simulink model "carsim_with_simulink3dof_open_loop_specific_control"  (R2023b)
settings: Solver=FixedStepAuto  StartTime=0.0  StopTime=25  FixedStep=0.001  RelTol=1e-3  EnableMultiTasking=on
values from neighbouring files (symbols this model uses):
  A = 5    [unlinear_vehicle_Parameters.m]
  Bf = 1.725    [unlinear_vehicle_Parameters.m]
  Br = 1.750    (= 1.75)    [unlinear_vehicle_Parameters.m]
  Cd = 0.4    [unlinear_vehicle_Parameters.m]
  Cs_f = 4302    [unlinear_vehicle_Parameters.m]
  Delta_act_sine_amp = delta_act_sine_amp(j)    [Truck_simulate.m]    (also in unlinear_vehicle_Parameters.m)
  Delta_act_sine_fre = delta_act_sine_fre(k)    [Truck_simulate.m]    (also in unlinear_vehicle_Parameters.m)
  f = 0.01    [unlinear_vehicle_Parameters.m]
  g = 9.8    [Truck_simulate.m]    (also in unlinear_vehicle_Parameters.m)
  He = 0.45    [unlinear_vehicle_Parameters.m]
  hg = 0.781    [unlinear_vehicle_Parameters.m]
  Hp = 0.2    [unlinear_vehicle_Parameters.m]
  I_tire = 0.7    [unlinear_vehicle_Parameters.m]
  Ix = 423.3    [unlinear_vehicle_Parameters.m]
  Iy = 1762.5    [unlinear_vehicle_Parameters.m]
  Iz = 1762.5    [unlinear_vehicle_Parameters.m]
  ks_f = 189000    [unlinear_vehicle_Parameters.m]
  kw = 220000    [unlinear_vehicle_Parameters.m]
  L = 3.140    (= 3.14)    [unlinear_vehicle_Parameters.m]
  Lf = 1.330    (= 1.33)    [unlinear_vehicle_Parameters.m]
  Lr = 3.140 - 1.330    (= 1.81)    [unlinear_vehicle_Parameters.m]
  m = m_sprung + m_load + m_unsprung    (= 10505)    [Truck_simulate.m]    (also in unlinear_vehicle_Parameters.m = 1407.3)
  mb = 1128.5 + 000    (= 1128.5)    [unlinear_vehicle_Parameters.m]
  mw = 139.4 / 2    (= 69.7)    [unlinear_vehicle_Parameters.m]
  p = 1.206    [unlinear_vehicle_Parameters.m]
  r = 0.510    (= 0.51)    [Truck_simulate.m]    (also in unlinear_vehicle_Parameters.m = 0.287)
  T_motor_constant = t_motor_const(i)    [Truck_simulate.m]    (also in unlinear_vehicle_Parameters.m)
  vx0 = 5    [Truck_simulate.m]    (also in unlinear_vehicle_Parameters.m)
  vy0 = 0    [Truck_simulate.m]    (also in unlinear_vehicle_Parameters.m)
  w0 = vx0 / r    (= 9.80392156863)    [Truck_simulate.m]    (also in unlinear_vehicle_Parameters.m = 17.4216027875)
  wz0 = 0    [Truck_simulate.m]    (also in unlinear_vehicle_Parameters.m)
libraries: Solver_SF x1
(part 1 of 4)
settings Model: Creator=dzY  LastModifiedBy=Admin
settings SolverCC: AlgebraicLoopSolver=TrustRegion
settings DataIOCC: SaveFormat=Array  ReturnWorkspaceOutputs=off
settings OptimizationCC: LifeSpan=inf
settings DebuggingCC: SolverPrmCheckMsg=warning  UnconnectedInputMsg=warning  UnconnectedOutputMsg=warning  UnconnectedLineMsg=warning  SFUnexpectedBacktrackingDiag=warning  SFNoUnconditionalDefaultTransitionDiag=warning  SFExecutionAtInitializationDiag=none  ArithmeticOperatorsInVariantConditions=warning
settings HardwareCC: ProdBitPerPointer=32  ProdBitPerSizeT=32  ProdBitPerPtrDiffT=32  ProdLargestAtomicFloat=None  ProdIntDivRoundTo=Undefined  ProdEndianess=Unspecified  ProdWordSize=32  ProdHWDeviceType=32-bit Generic
settings ModelReferenceCC: EnableRefExpFcnMdlSchedulingChecks=on  PropagateSignalLabelsOutOfModel=off
settings SFSimCC: SimUseLocalCustomCode=off  CustomCodeUndefinedFunction=UseInterfaceOnly
settings RTWCC: RTWUseLocalCustomCode=off
settings CodeAppCC: StateflowObjectComments=on
settings GRTTargetCC: TargetLangStandard=C89/C90 (ANSI)
settings ConfigComp: CovMetricSettings=dw  CovSaveCumulativeToWorkspaceVar=on  CovSaveSingleToWorkspaceVar=on  CovExternalEMLEnable=off  CovSFcnEnable=off

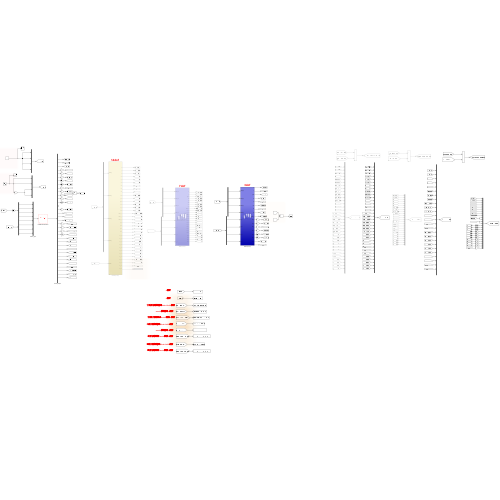
[thumbnail: Simulink's stored preview of the top-level diagram]
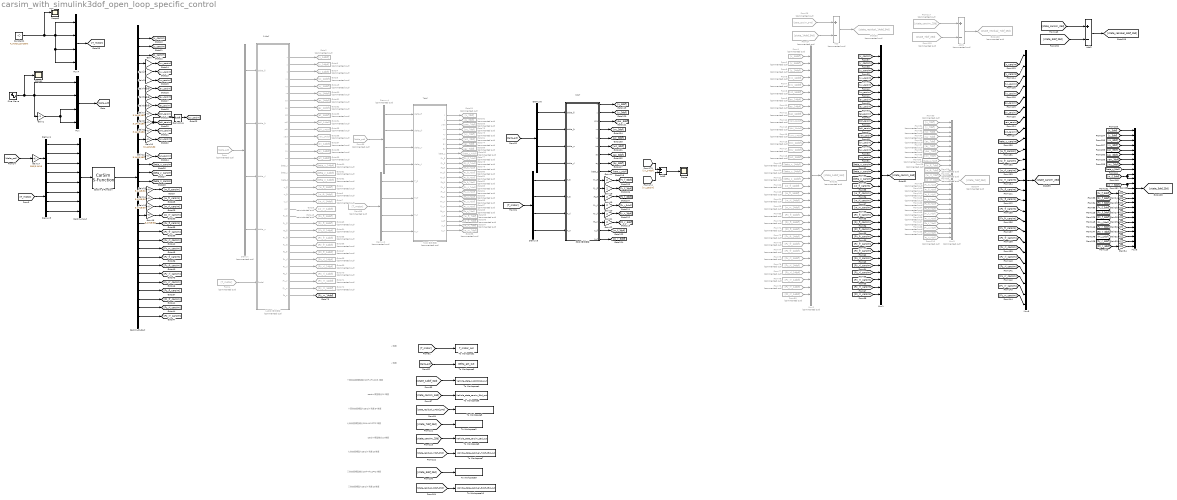
== system carsim_with_simulink3dof_open_loop_specific_control ==
  note: 7dof
  note: 4维度
  note: 4维度
  note: 十四自由度模型输出18+4+12=34维度
  note: carsim模型输出34维度
  note: 十四自由度模型与carsim残差34维度
  note: carsim模型输出25维度
  note: 七自由度模型与carsim残差25维度
  note: 七自由度模型输出18+4+12=25维度
  note: 14dof
  note: 3dof
  note: 三自由度模型与carsim残差25维度
  note: 三自由度模型输出18+4+12=25维度
  14DOF整车模型 : Subsystem  Commented=on
  3DOF整车模型 : Subsystem
  7DOF整车模型 : Subsystem  Commented=on
  Add : Sum  Commented=on  Inputs=+-
  Add1 : Sum  Commented=on  Inputs=+-
  Add2 : Sum  Inputs=+-
  Add3 : Sum  Inputs=+-
  CarSim S-Function : Solver_SF/CarSim S-Function  Priority=1  SIMFILE=simfile.sim  Run_RTs=off  vs_state_ind=Run  StopMode_ind=Vehicle Model
  Carsim_Input : Mux  Inputs=8
  Carsim_Output : Demux  Outputs=34
  Constant1 : Constant  Value=T_motor_constant
  Demux : Demux  Commented=on
  Demux{1,3,5..6} (4 alike) : Demux
  Demux2 : Demux  Commented=on
  Demux4 : Demux  Commented=on
  Derivative : Derivative
  From : From  Commented=on  GotoTag=delta_act
  From1 : From  Commented=on  GotoTag=x_14dof
  From10 : From  Commented=on  GotoTag=ay_14dof
  From100 : From  Commented=on  GotoTag=Fy_fl_7dof
  From101 : From  Commented=on  GotoTag=Fz_fl_7dof
  From102 : From  Commented=on  GotoTag=Fx_fr_7dof
  From103 : From  Commented=on  GotoTag=Fy_fr_7dof
  From104 : From  Commented=on  GotoTag=Fz_fr_7dof
  From105 : From  Commented=on  GotoTag=Fx_rl_7dof
  From106 : From  Commented=on  GotoTag=Fy_rl_7dof
  From107 : From  Commented=on  GotoTag=Fz_rl_7dof
  From108 : From  Commented=on  GotoTag=Fx_rr_7dof
  From109 : From  Commented=on  GotoTag=Fy_rr_7dof
  From11 : From  Commented=on  GotoTag=az_14dof
  From110 : From  Commented=on  GotoTag=Fz_rr_7dof
  From115 : From  Commented=on  GotoTag=state_7dof_25d
  From117 : From  Commented=on  GotoTag=state_carsim_25d
  From12 : From  Commented=on  GotoTag=roll_14dof
  From13 : From  Commented=on  GotoTag=phi_14dof
  From15 : From  Commented=on  GotoTag=yaw_14dof
  From16 : From  Commented=on  GotoTag=wx_14dof
  From17 : From  Commented=on  GotoTag=wy_14dof
  From18 : From  Commented=on  GotoTag=wz_14dof
  From19 : From  Commented=on  GotoTag=beta_x_14dof
  From2 : From  Commented=on  GotoTag=y_14dof
  From20 : From  Commented=on  GotoTag=beta_y_14dof
  From21 : From  Commented=on  GotoTag=beta_z_14dof
  From22 : From  Commented=on  GotoTag=w_fl_14dof
  From23 : From  Commented=on  GotoTag=w_fr_14dof
  From24 : From  Commented=on  GotoTag=w_rl_14dof
  From25 : From  Commented=on  GotoTag=w_rr_14dof
  From26 : From  Commented=on  GotoTag=state_carsim_34d
  From27 : From  Commented=on  GotoTag=state_14dof_34d
  From28 : From  Commented=on  GotoTag=w_fl_7dof
  From29 : From  Commented=on  GotoTag=w_fr_7dof
  From30 : From  Commented=on  GotoTag=w_rl_7dof
  From4 : From  Commented=on  GotoTag=T_motor
  From5 : From  Commented=on  GotoTag=z_14dof
  From6 : From  Commented=on  GotoTag=vx_14dof
  From69 : From  Commented=on  GotoTag=Fx_fl_14dof
  From7 : From  Commented=on  GotoTag=vy_14dof
  From70 : From  Commented=on  GotoTag=Fy_fl_14dof
  From71 : From  Commented=on  GotoTag=Fz_fl_14dof
  From72 : From  Commented=on  GotoTag=Fx_fr_14dof
  From73 : From  Commented=on  GotoTag=Fy_fr_14dof
  From74 : From  Commented=on  GotoTag=Fz_fr_14dof
  From75 : From  Commented=on  GotoTag=Fx_rl_14dof
  From76 : From  Commented=on  GotoTag=Fy_rl_14dof
  From77 : From  Commented=on  GotoTag=Fz_rl_14dof
  From78 : From  Commented=on  GotoTag=Fx_rr_14dof
  From79 : From  Commented=on  GotoTag=Fy_rr_14dof
  From8 : From  Commented=on  GotoTag=vz_14dof
  From80 : From  Commented=on  GotoTag=Fz_rr_14dof
  From85 : From  Commented=on  GotoTag=w_rr_7dof
  From88 : From  Commented=on  GotoTag=T_motor
  From89 : From  Commented=on  GotoTag=delta_act
  From9 : From  Commented=on  GotoTag=ax_14dof
  From90 : From  Commented=on  GotoTag=x_7dof
  From91 : From  Commented=on  GotoTag=y_7dof
  From92 : From  Commented=on  GotoTag=yaw_7dof
  From93 : From  Commented=on  GotoTag=vx_7dof
  From94 : From  Commented=on  GotoTag=vy_7dof
  From95 : From  Commented=on  GotoTag=wz_7dof
  From96 : From  Commented=on  GotoTag=ax_7dof
  From97 : From  Commented=on  GotoTag=ay_7dof
  From98 : From  Commented=on  GotoTag=beta_z_7dof
  From99 : From  Commented=on  GotoTag=Fx_fl_7dof
  Gain : Gain  Gain=1/3.6
  Gain1 : Gain  Gain=-1
  Gain{7..10,12} (5 alike) : Gain  Gain=3.1415/180
  Gain{11,18..22} (6 alike) : Gain  Gain=2
  Gain{13..16} (4 alike) : Gain  Gain=3.1415/30
  Gain17 : Gain  Gain=180/3.1415
  Gain2 : Gain  Gain=1/3.6
  Gain{23..34} (12 alike) : Gain  Gain=0.5
  Gain3 : Gain  Gain=1/3.6
  Gain4 : Gain  Gain=9.8
  Gain5 : Gain  Gain=9.8
  Gain6 : Gain  Gain=9.8
  Goto1 : Goto  Commented=on  GotoTag=w_fl_14dof
  Goto100 : Goto  Commented=on  GotoTag=state_residual_7dof_25d
  Goto2 : Goto  Commented=on  GotoTag=x_14dof
  Goto3 : Goto  Commented=on  GotoTag=y_14dof
  Goto32 : Goto  Commented=on  GotoTag=state_14dof_34d
  Goto33 : Goto  Commented=on  GotoTag=state_residual_14dof_34d
  Goto34 : Goto  Commented=on  GotoTag=wz_7dof
  Goto4 : Goto  Commented=on  GotoTag=z_14dof
  Goto48 : Goto  Commented=on  GotoTag=Fx_fl_14dof
  Goto49 : Goto  Commented=on  GotoTag=vy_14dof
  Goto5 : Goto  Commented=on  GotoTag=vx_14dof
  Goto50 : Goto  Commented=on  GotoTag=vz_14dof
  Goto51 : Goto  Commented=on  GotoTag=ax_14dof
  Goto52 : Goto  Commented=on  GotoTag=ay_14dof
  Goto53 : Goto  Commented=on  GotoTag=az_14dof
  Goto54 : Goto  Commented=on  GotoTag=roll_14dof
  Goto55 : Goto  Commented=on  GotoTag=phi_14dof
  Goto56 : Goto  Commented=on  GotoTag=yaw_14dof
  Goto57 : Goto  Commented=on  GotoTag=wx_14dof
  Goto58 : Goto  Commented=on  GotoTag=wy_14dof
  Goto59 : Goto  Commented=on  GotoTag=wz_14dof
  Goto6 : Goto  Commented=on  GotoTag=w_fr_14dof
  Goto60 : Goto  Commented=on  GotoTag=beta_x_14dof
  Goto61 : Goto  Commented=on  GotoTag=beta_y_14dof
  Goto62 : Goto  Commented=on  GotoTag=beta_z_14dof
  Goto63 : Goto  Commented=on  GotoTag=Fy_fl_14dof
  Goto64 : Goto  Commented=on  GotoTag=Fz_fl_14dof
  Goto65 : Goto  Commented=on  GotoTag=Fx_fr_14dof
  Goto66 : Goto  Commented=on  GotoTag=Fy_fr_14dof
  Goto67 : Goto  Commented=on  GotoTag=Fz_fr_14dof
  Goto68 : Goto  Commented=on  GotoTag=Fx_rl_14dof
  Goto69 : Goto  Commented=on  GotoTag=Fy_rl_14dof
  Goto7 : Goto  Commented=on  GotoTag=w_rl_14dof
  Goto70 : Goto  Commented=on  GotoTag=Fz_rl_14dof
  Goto71 : Goto  Commented=on  GotoTag=Fx_rr_14dof
  Goto72 : Goto  Commented=on  GotoTag=Fy_rr_14dof
  Goto74 : Goto  Commented=on  GotoTag=ax_7dof
  Goto75 : Goto  Commented=on  GotoTag=vy_7dof
  Goto76 : Goto  Commented=on  GotoTag=vx_7dof
  Goto77 : Goto  Commented=on  GotoTag=Fx_fl_7dof
  Goto78 : Goto  Commented=on  GotoTag=Fy_fl_7dof
  Goto79 : Goto  Commented=on  GotoTag=Fz_fl_7dof
  Goto8 : Goto  Commented=on  GotoTag=w_rr_14dof
  Goto80 : Goto  Commented=on  GotoTag=Fx_fr_7dof
  Goto81 : Goto  Commented=on  GotoTag=Fy_fr_7dof
  Goto82 : Goto  Commented=on  GotoTag=Fz_fr_7dof
  Goto83 : Goto  Commented=on  GotoTag=Fx_rl_7dof
  Goto84 : Goto  Commented=on  GotoTag=Fy_rl_7dof
  Goto85 : Goto  Commented=on  GotoTag=Fz_rl_7dof
  Goto86 : Goto  Commented=on  GotoTag=Fx_rr_7dof
  Goto87 : Goto  Commented=on  GotoTag=Fy_rr_7dof
  Goto88 : Goto  Commented=on  GotoTag=Fz_rr_7dof
  Goto89 : Goto  Commented=on  GotoTag=ay_7dof
  Goto90 : Goto  Commented=on  GotoTag=beta_z_7dof
  Goto91 : Goto  Commented=on  GotoTag=x_7dof
  Goto92 : Goto  Commented=on  GotoTag=y_7dof
  Goto93 : Goto  Commented=on  GotoTag=yaw_7dof
  Goto94 : Goto  Commented=on  GotoTag=state_7dof_25d
  Goto95 : Goto  Commented=on  GotoTag=w_fl_7dof
  Goto96 : Goto  Commented=on  GotoTag=w_fr_7dof
  Goto97 : Goto  Commented=on  GotoTag=w_rl_7dof
  Goto98 : Goto  Commented=on  GotoTag=w_rr_7dof
  Mux : Mux
  Mux1 : Mux  Inputs=34
  Mux2 : Mux  Commented=on  Inputs=34
  Mux3 : Mux  Commented=on  Inputs=25
  Mux4 : Mux
  Mux5 : Mux  Inputs=25
  Mux6 : Mux  Inputs=25
  Scope : Scope
  Scope4 : Scope
  Scope5 : Scope
  Sine Wave : Sin  Amplitude=Delta_act_sine_amp  Frequency=Delta_act_sine_fre  SampleTime=0
  To Workspace1 : ToWorkspace  VariableName=T_motor_out  SaveFormat=Timeseries  SampleTime=-1
  To Workspace10 : ToWorkspace  VariableName=Vehicle_state_residual_3dof_25d_out  SaveFormat=Timeseries  SampleTime=-1
  To Workspace2 : ToWorkspace  VariableName=Vehicle_state_7dof_25d_out  SaveFormat=Timeseries  SampleTime=-1
  To Workspace3 : ToWorkspace  VariableName=Delta_act_out  SaveFormat=Timeseries  SampleTime=-1
  To Workspace4 : ToWorkspace  VariableName=Vehicle_state_14dof_34d_out  SaveFormat=Timeseries  SampleTime=-1
  To Workspace5 : ToWorkspace  VariableName=Vehicle_state_residual_14dof_34d_out  SaveFormat=Timeseries  SampleTime=-1
  To Workspace6 : ToWorkspace  VariableName=Vehicle_state_carsim_34d_out  SaveFormat=Timeseries  SampleTime=-1
  To Workspace7 : ToWorkspace  VariableName=Vehicle_state_residual_7dof_25d_out  SaveFormat=Timeseries  SampleTime=-1
  To Workspace8 : ToWorkspace  VariableName=Vehicle_state_carsim_25d_out  SaveFormat=Timeseries  SampleTime=-1
  To Workspace9 : ToWorkspace  VariableName=Vehicle_state_3dof_25d_out  SaveFormat=Timeseries  SampleTime=-1
  wires:
  From4/1 -> 14DOF整车模型/5(Pedal)
  Mux4/1 -> [T_motor]
  Constant1/1 -> Mux4/1, Mux4/4, Mux4/3, Mux4/2, Scope5/1
  Carsim_Input/1 -> CarSim S-Function/1
  CarSim S-Function/1 -> Carsim_Output/1
  [T_motor] -> Demux3/1
  Demux3/1 -> Carsim_Input/5
  Demux3/2 -> Carsim_Input/6
  Demux3/3 -> Carsim_Input/7
  Demux3/4 -> Carsim_Input/8
  14DOF整车模型/1(x) -> Goto2/1
  14DOF整车模型/2(y) -> Goto3/1
  14DOF整车模型/3(z) -> Goto4/1
  14DOF整车模型/4(vx) -> Goto5/1
  14DOF整车模型/5(vy) -> Goto49/1
  14DOF整车模型/6(vz) -> Goto50/1
  14DOF整车模型/7(ax) -> Goto51/1
  14DOF整车模型/8(ay) -> Goto52/1
  14DOF整车模型/9(az) -> Goto53/1
  14DOF整车模型/10(roll) -> Goto54/1
  14DOF整车模型/11(phi) -> Goto55/1
  14DOF整车模型/12(yaw) -> Goto56/1
  14DOF整车模型/13(wx) -> Goto57/1
  14DOF整车模型/14(wy) -> Goto58/1
  14DOF整车模型/15(wz) -> Goto59/1
  14DOF整车模型/16(beta_x) -> Goto60/1
  14DOF整车模型/17(beta_y) -> Goto61/1
  14DOF整车模型/18(beta_z) -> Goto62/1
  From1/1 -> Mux2/1
  From2/1 -> Mux2/2
  From5/1 -> Mux2/3
  From6/1 -> Mux2/4
  From7/1 -> Mux2/5
  From8/1 -> Mux2/6
  From9/1 -> Mux2/7
  From10/1 -> Mux2/8
  From11/1 -> Mux2/9
  From12/1 -> Mux2/10
  From13/1 -> Mux2/11
  From15/1 -> Mux2/12
  From16/1 -> Mux2/13
  From17/1 -> Mux2/14
  From18/1 -> Mux2/15
  From19/1 -> Mux2/16
  From20/1 -> Mux2/17
  From21/1 -> Mux2/18
  Mux2/1 -> Goto32/1
  Sine Wave/1 -> Mux/1, Mux/2, Gain1/1, Scope4/1
  Mux/1 -> [delta_act]
  Gain1/1 -> Mux/4, Mux/3
  Demux/4 -> 14DOF整车模型/4(delta_rr)
  Demux/3 -> 14DOF整车模型/3(delta_rl)
  Demux/2 -> 14DOF整车模型/2(delta_fr)
  Demux/1 -> 14DOF整车模型/1(delta_fl)
  From/1 -> Demux/1
  Demux1/4 -> Carsim_Input/4
  Demux1/3 -> Carsim_Input/3
  Demux1/2 -> Carsim_Input/2
  Demux1/1 -> Carsim_Input/1
  14DOF整车模型/19(w_fl) -> Goto1/1
  14DOF整车模型/20(w_fr) -> Goto6/1
  14DOF整车模型/21(w_rl) -> Goto7/1
  14DOF整车模型/22(wrr) -> Goto8/1
  From22/1 -> Mux2/19
  From23/1 -> Mux2/20
  From24/1 -> Mux2/21
  From25/1 -> Mux2/22
  Carsim_Output/2 -> [y_carsim]
  Carsim_Output/1 -> [x_carsim]
  Carsim_Output/3 -> [z_carsim]
  Carsim_Output/16 -> [beta_x_carsim]
  Carsim_Output/17 -> [beta_y_carsim]
  Carsim_Output/18 -> [beta_z_carsim]
  From27/1 -> Add/2
  From26/1 -> Add/1
  Add/1 -> Goto33/1
  Carsim_Output/6 -> Gain3/1
  Gain3/1 -> [vz_carsim]
  Carsim_Output/5 -> Gain2/1
  Gain2/1 -> [vy_carsim]
  Gain/1 -> [vx_carsim]
  Carsim_Output/4 -> Gain/1
  Carsim_Output/7 -> Gain4/1
  Gain4/1 -> [ax_carsim]
  Carsim_Output/8 -> Gain5/1
  Gain5/1 -> [ay_carsim]
  Carsim_Output/9 -> Gain6/1
  Gain6/1 -> [az_carsim]
  Carsim_Output/10 -> Gain7/1
  Gain7/1 -> [roll_carsim]
  Carsim_Output/11 -> Gain8/1
  Gain8/1 -> Derivative/1, [phi_carsim]
  Carsim_Output/12 -> Gain9/1
  Gain9/1 -> [yaw_carsim]
  Carsim_Output/15 -> Gain12/1
  Carsim_Output/13 -> Gain10/1
  Gain10/1 -> [wx_carsim]
  Gain12/1 -> [wz_carsim]
  Carsim_Output/19 -> Gain13/1
  Gain13/1 -> [w_fl_carsim]
  Carsim_Output/20 -> Gain14/1
  Gain14/1 -> [w_fr_carsim]
  Carsim_Output/21 -> Gain15/1
  Carsim_Output/22 -> Gain16/1
  Gain15/1 -> [w_rl_carsim]
  Gain16/1 -> [w_rr_carsim]
  Gain17/1 -> Demux1/1
  [delta_act] -> Gain17/1
  Derivative/1 -> [wy_carsim]
  [x_carsim] -> Mux1/1
  [y_carsim] -> Mux1/2
  [z_carsim] -> Mux1/3
  [vx_carsim] -> Mux1/4
  [vy_carsim] -> Mux1/5
  [vz_carsim] -> Mux1/6
  [ax_carsim] -> Mux1/7
  [ay_carsim] -> Mux1/8
  [az_carsim] -> Mux1/9
  [roll_carsim] -> Mux1/10
  [phi_carsim] -> Mux1/11
  [yaw_carsim] -> Mux1/12
  [wx_carsim] -> Mux1/13
  [wy_carsim] -> Mux1/14
  [wz_carsim] -> Mux1/15
  [beta_x_carsim] -> Mux1/16
  [beta_y_carsim] -> Mux1/17
  [beta_z_carsim] -> Mux1/18
  [w_fl_carsim] -> Mux1/19
  [w_fr_carsim] -> Mux1/20
  [w_rl_carsim] -> Mux1/21
  [w_rr_carsim] -> Mux1/22
  Mux1/1 -> [state_carsim_34d]
  [Fx_fl_carsim] -> Mux1/23
  [Fy_fl_carsim] -> Mux1/24
  [Fz_fl_carsim] -> Mux1/25
  [Fx_fr_carsim] -> Mux1/26
  [Fy_fr_carsim] -> Mux1/27
  [Fz_fr_carsim] -> Mux1/28
  [Fx_rl_carsim] -> Mux1/29
  [Fy_rl_carsim] -> Mux1/30
  [Fz_rl_carsim] -> Mux1/31
  [Fx_rr_carsim] -> Mux1/32
  [Fy_rr_carsim] -> Mux1/33
  [Fz_rr_carsim] -> Mux1/34
  14DOF整车模型/23(Fx_fl) -> Goto48/1
  14DOF整车模型/24(Fy_fl) -> Goto63/1
  14DOF整车模型/25(Fz_fl) -> Goto64/1
  14DOF整车模型/26(Fx_fr) -> Goto65/1
  14DOF整车模型/27(Fy_fr) -> Goto66/1
  14DOF整车模型/28(Fz_fr) -> Goto67/1
  14DOF整车模型/29(Fx_rl) -> Goto68/1
  14DOF整车模型/30(Fy_rl) -> Goto69/1
  14DOF整车模型/31(Fz_rl) -> Goto70/1
  14DOF整车模型/32(Fx_rr) -> Goto71/1
  14DOF整车模型/33(Fy_rr) -> Goto72/1
  14DOF整车模型/34(Fz_rr) -> [Fz_rr_14dof]
  From69/1 -> Mux2/23
  From70/1 -> Mux2/24
  From71/1 -> Mux2/25
  From72/1 -> Mux2/26
  From73/1 -> Mux2/27
  From74/1 -> Mux2/28
  From75/1 -> Mux2/29
  From76/1 -> Mux2/30
  From77/1 -> Mux2/31
  From78/1 -> Mux2/32
  From79/1 -> Mux2/33
  From80/1 -> Mux2/34
  [T_motor] -> To Workspace1/1
  [delta_act] -> To Workspace3/1
  [state_14dof_34d] -> To Workspace4/1
  [state_residual_14dof_34d] -> To Workspace5/1
  Carsim_Output/23 -> [Fx_fl_carsim]
  Carsim_Output/24 -> [Fx_fr_carsim]
  Carsim_Output/25 -> [Fx_rl_carsim]
  Carsim_Output/26 -> [Fx_rr_carsim]
  Carsim_Output/27 -> [Fy_fl_carsim]
  Carsim_Output/28 -> [Fy_fr_carsim]
  Carsim_Output/29 -> [Fy_rl_carsim]
  Carsim_Output/30 -> [Fy_rr_carsim]
  Carsim_Output/31 -> [Fz_fl_carsim]
  Carsim_Output/32 -> [Fz_fr_carsim]
  Carsim_Output/33 -> [Fz_rl_carsim]
  Carsim_Output/34 -> [Fz_rr_carsim]
  7DOF整车模型/17(Fy_rl) -> Goto84/1
  7DOF整车模型/10(Fx_fl) -> Goto77/1
  7DOF整车模型/19(Fx_rr) -> Goto86/1
  7DOF整车模型/21(Fz_rr) -> Goto88/1
  7DOF整车模型/14(Fy_fr) -> Goto81/1
  7DOF整车模型/11(Fy_fl) -> Goto78/1
  7DOF整车模型/12(Fz_fl) -> Goto79/1
  7DOF整车模型/20(Fy_rr) -> Goto87/1
  7DOF整车模型/13(Fx_fr) -> Goto80/1
  7DOF整车模型/18(Fz_rl) -> Goto85/1
  7DOF整车模型/16(Fx_rl) -> Goto83/1
  7DOF整车模型/15(Fz_fr) -> Goto82/1
  From88/1 -> Demux2/1
  Demux2/1 -> 7DOF整车模型/5(T_fl)
  Demux2/2 -> 7DOF整车模型/6(T_fr)
  Demux2/3 -> 7DOF整车模型/7(T_rl)
  Demux2/4 -> 7DOF整车模型/8(T_rr)
  Demux4/1 -> 7DOF整车模型/1(delta_fl)
  Demux4/2 -> 7DOF整车模型/2(delta_fr)
  Demux4/3 -> 7DOF整车模型/3(delta_rr)
  Demux4/4 -> 7DOF整车模型/4(delta_rl)
  From89/1 -> Demux4/1
  7DOF整车模型/9(beta_z) -> Goto90/1
  7DOF整车模型/8(ay) -> Goto89/1
  7DOF整车模型/1(x) -> Goto91/1
  7DOF整车模型/2(y) -> Goto92/1
  7DOF整车模型/3(yaw) -> Goto93/1
  7DOF整车模型/4(vx) -> Goto76/1
  7DOF整车模型/5(vy) -> Goto75/1
  7DOF整车模型/6(wz) -> Goto34/1
  7DOF整车模型/7(ax) -> Goto74/1
  From90/1 -> Mux3/1
  From91/1 -> Mux3/2
  Mux3/1 -> Goto94/1
  [state_carsim_34d] -> To Workspace6/1
  7DOF整车模型/22(w_fl) -> Goto95/1
  7DOF整车模型/23(w_fr) -> Goto96/1
  7DOF整车模型/24(w_rl) -> Goto97/1
  7DOF整车模型/25(w_rr) -> Goto98/1
  From28/1 -> Mux3/10
  From29/1 -> Mux3/11
  From30/1 -> Mux3/12
  From85/1 -> Mux3/13
  From99/1 -> Mux3/14
  From100/1 -> Mux3/15
  From101/1 -> Mux3/16
  From102/1 -> Mux3/17
  From103/1 -> Mux3/18
  From104/1 -> Mux3/19
  From105/1 -> Mux3/20
  From106/1 -> Mux3/21
  From107/1 -> Mux3/22
  From108/1 -> Mux3/23
  From109/1 -> Mux3/24
  From110/1 -> Mux3/25
  Mux5/1 -> [state_carsim_25d]
  [x_carsim] -> Mux5/1
  [y_carsim] -> Mux5/2
  [vx_carsim] -> Mux5/3
  [vy_carsim] -> Mux5/4
  [ax_carsim] -> Mux5/5
  [ay_carsim] -> Mux5/6
  [yaw_carsim] -> Mux5/7
  [wz_carsim] -> Mux5/8
  [beta_z_carsim] -> Mux5/9
  [w_fl_carsim] -> Mux5/10
  [w_fr_carsim] -> Mux5/11
  [w_rl_carsim] -> Mux5/12
  [w_rr_carsim] -> Mux5/13
  [Fx_fl_carsim] -> Mux5/14
  [Fy_fl_carsim] -> Mux5/15
  [Fz_fl_carsim] -> Mux5/16
  [Fx_fr_carsim] -> Mux5/17
  [Fy_fr_carsim] -> Mux5/18
  [Fz_fr_carsim] -> Mux5/19
  [Fx_rl_carsim] -> Mux5/20
  [Fy_rl_carsim] -> Mux5/21
  [Fz_rl_carsim] -> Mux5/22
  [Fx_rr_carsim] -> Mux5/23
  [Fy_rr_carsim] -> Mux5/24
  [Fz_rr_carsim] -> Mux5/25
  From98/1 -> Mux3/9
  From95/1 -> Mux3/8
  From92/1 -> Mux3/7
  From97/1 -> Mux3/6
  From96/1 -> Mux3/5
  From94/1 -> Mux3/4
  From93/1 -> Mux3/3
  From117/1 -> Add1/1
  From115/1 -> Add1/2
  Add1/1 -> Goto100/1
  [state_carsim_25d] -> To Workspace8/1
  [state_7dof_25d] -> To Workspace2/1
  [state_residual_7dof_25d] -> To Workspace7/1
  3DOF整车模型/17(w_rl) -> [w_r_3dof]
  Demux5/1 -> 3DOF整车模型/5(T_fl)
  3DOF整车模型/9(beta_z) -> [beta_z_3dof]
  3DOF整车模型/4(vx) -> [vx_3dof]
  Demux5/2 -> 3DOF整车模型/6(T_fr)
  [delta_act] -> Demux6/1
  3DOF整车模型/6(wz) -> [wz_3dof]
  Demux6/3 -> 3DOF整车模型/3(delta_rr)
  3DOF整车模型/8(ay) -> [ay_3dof]
  Demux6/1 -> 3DOF整车模型/1(delta_fl)
  3DOF整车模型/16(w_fl) -> [w_f_3dof]
  3DOF整车模型/3(yaw) -> [yaw_3dof]
  3DOF整车模型/5(vy) -> [vy_3dof]
  Demux5/3 -> 3DOF整车模型/7(T_rl)
  3DOF整车模型/7(ax) -> [ax_3dof]
  [T_motor] -> Demux5/1
  3DOF整车模型/1(x) -> [x_3dof]
  Demux6/4 -> 3DOF整车模型/4(delta_rl)
  Demux6/2 -> 3DOF整车模型/2(delta_fr)
  Demux5/4 -> 3DOF整车模型/8(T_rr)
  3DOF整车模型/2(y) -> [y_3dof]
  3DOF整车模型/10(Fx_fl) -> Gain11/1
  Gain11/1 -> [Fx_f_3dof]
  3DOF整车模型/11(Fy_fl) -> Gain18/1
  Gain18/1 -> [Fy_f_3dof]
  3DOF整车模型/12(Fz_fl) -> Gain19/1
  Gain19/1 -> [Fz_f_3dof]
  3DOF整车模型/13(Fx_rl) -> Gain20/1
  Gain20/1 -> [Fx_r_3dof]
  3DOF整车模型/14(Fy_rl) -> Gain21/1
  Gain21/1 -> [Fy_r_3dof]
  3DOF整车模型/15(Fz_rl) -> Gain22/1
  Gain22/1 -> [Fz_r_3dof]
  [beta_z_3dof] -> Mux6/9
  [vx_3dof] -> Mux6/3
  [vy_3dof] -> Mux6/4
  [ay_3dof] -> Mux6/6
  [yaw_3dof] -> Mux6/7
  [ax_3dof] -> Mux6/5
  [wz_3dof] -> Mux6/8
  [y_3dof] -> Mux6/2
  Mux6/1 -> [state_3dof_25d]
  [x_3dof] -> Mux6/1
  [w_f_3dof] -> Mux6/10, Mux6/11
  [w_r_3dof] -> Mux6/12, Mux6/13
  [Fx_f_3dof] -> Gain23/1
  Gain23/1 -> Mux6/14
  [Fy_f_3dof] -> Gain24/1
  Gain24/1 -> Mux6/15
  Gain25/1 -> Mux6/16
  [Fz_f_3dof] -> Gain25/1
  [Fx_f_3dof] -> Gain26/1
  [Fz_f_3dof] -> Gain28/1
  [Fy_f_3dof] -> Gain27/1
  Gain26/1 -> Mux6/17
  Gain27/1 -> Mux6/18
  Gain28/1 -> Mux6/19
  [Fx_r_3dof] -> Gain29/1
  [Fx_r_3dof] -> Gain32/1
  [Fz_r_3dof] -> Gain31/1
  [Fz_r_3dof] -> Gain34/1
  [Fy_r_3dof] -> Gain30/1
  [Fy_r_3dof] -> Gain33/1
  Gain30/1 -> Mux6/21
  Gain29/1 -> Mux6/20
  Gain32/1 -> Mux6/23
  Gain33/1 -> Mux6/24
  Gain31/1 -> Mux6/22
  Gain34/1 -> Mux6/25
  [state_3dof_25d] -> Add2/2
  [state_carsim_25d] -> Add2/1
  Add2/1 -> [state_residual_3dof_25d]
  [state_residual_3dof_25d] -> To Workspace10/1
  [state_3dof_25d] -> To Workspace9/1
  [vx_14dof] -> Add3/1
  [vx_carsim] -> Add3/2
  Add3/1 -> Scope/1

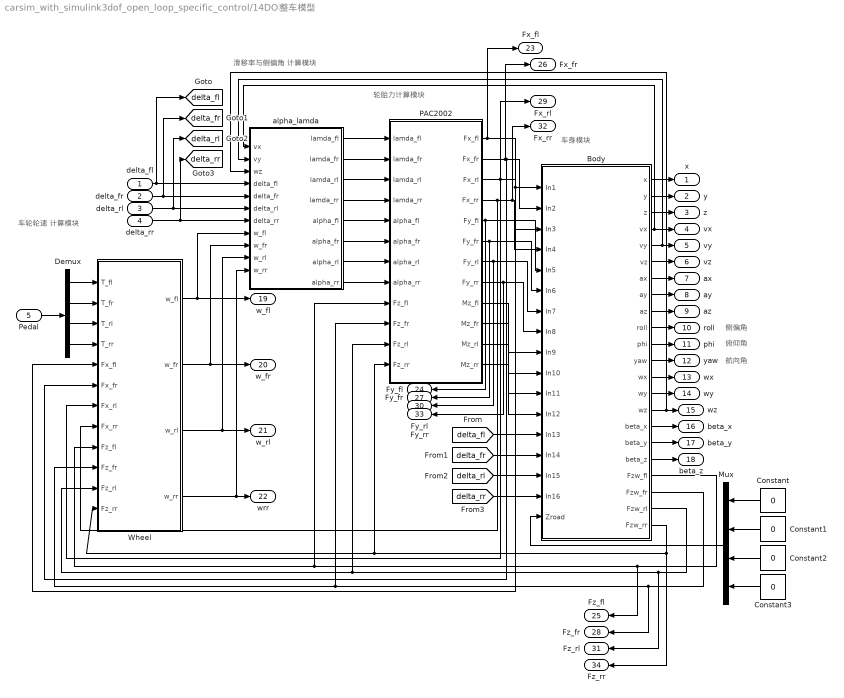
== system carsim_with_simulink3dof_open_loop_specific_control/14DOF整车模型 ==
  note: 车身模块
  note: 航向角
  note: 侧偏角
  note: 俯仰角
  note: 轮胎力计算模块
  note: 滑移率与侧偏角
      | 计算模块
  note: 车轮轮速
      | 计算模块
  delta_fl : Inport
  delta_fr : Inport  Port=2
  delta_rl : Inport  Port=3
  delta_rr : Inport  Port=4
  Pedal : Inport  Port=5
  Body : Subsystem
  Constant{,1..3} (4 alike) : Constant  Value=0
  Demux : Demux
  Mux : Mux
  PAC2002 : Subsystem
  Wheel : Subsystem
  alpha_lamda : Subsystem
  x : Outport
  y : Outport  Port=2
  z : Outport  Port=3
  vx : Outport  Port=4
  vy : Outport  Port=5
  vz : Outport  Port=6
  ax : Outport  Port=7
  ay : Outport  Port=8
  az : Outport  Port=9
  roll : Outport  Port=10
  phi : Outport  Port=11
  yaw : Outport  Port=12
  wx : Outport  Port=13
  wy : Outport  Port=14
  wz : Outport  Port=15
  beta_x : Outport  Port=16
  beta_y : Outport  Port=17
  beta_z : Outport  Port=18
  w_fl : Outport  Port=19
  w_fr : Outport  Port=20
  w_rl : Outport  Port=21
  wrr : Outport  Port=22
  Fx_fl : Outport  Port=23
  Fy_fl : Outport  Port=24
  Fz_fl : Outport  Port=25
  Fx_fr : Outport  Port=26
  Fy_fr : Outport  Port=27
  Fz_fr : Outport  Port=28
  Fx_rl : Outport  Port=29
  Fy_rl : Outport  Port=30
  Fz_rl : Outport  Port=31
  Fx_rr : Outport  Port=32
  Fy_rr : Outport  Port=33
  Fz_rr : Outport  Port=34
  tag scope: delta_fl=global, delta_fr=global, delta_rl=global, delta_rr=global
  wires:
  delta_fl/1 -> alpha_lamda/4(delta_fl), [delta_fl]
  delta_rr/1 -> alpha_lamda/7(delta_rr), [delta_rr]
  delta_fr/1 -> alpha_lamda/5(delta_fr), [delta_fr]
  delta_rl/1 -> [delta_rl], alpha_lamda/6(delta_rl)
  alpha_lamda/1(lamda_fl) -> PAC2002/1(lamda_fl)
  alpha_lamda/7(alpha_rl) -> PAC2002/7(alpha_rl)
  Wheel/2(w_fr) -> w_fr/1, alpha_lamda/9(w_fr)
  PAC2002/5(Fy_fl) -> Body/5(In5), Fy_fl/1
  alpha_lamda/2(lamda_fr) -> PAC2002/2(lamda_fr)
  alpha_lamda/5(alpha_fl) -> PAC2002/5(alpha_fl)
  alpha_lamda/3(lamda_rl) -> PAC2002/3(lamda_rl)
  alpha_lamda/4(lamda_rr) -> PAC2002/4(lamda_rr)
  PAC2002/9(Mz_fl) -> Body/9(In9)
  PAC2002/10(Mz_fr) -> Body/10(In10)
  Wheel/4(w_rr) -> alpha_lamda/11(w_rr), wrr/1
  PAC2002/4(Fx_rr) -> Fx_rr/1, Body/4(In4), Wheel/8(Fx_rr)
  alpha_lamda/6(alpha_fr) -> PAC2002/6(alpha_fr)
  PAC2002/3(Fx_rl) -> Fx_rl/1, Body/3(In3), Wheel/7(Fx_rl)
  Wheel/3(w_rl) -> w_rl/1, alpha_lamda/10(w_rl)
  PAC2002/7(Fy_rl) -> Fy_rl/1, Body/7(In7)
  PAC2002/2(Fx_fr) -> Body/2(In2), Wheel/6(Fx_fr), Fx_fr/1
  PAC2002/8(Fy_rr) -> Fy_rr/1, Body/8(In8)
  alpha_lamda/8(alpha_rr) -> PAC2002/8(alpha_rr)
  PAC2002/1(Fx_fl) -> Wheel/5(Fx_fl), Body/1(In1), Fx_fl/1
  PAC2002/12(Mz_rr) -> Body/12(In12)
  Demux/3 -> Wheel/3(T_rl)
  Demux/2 -> Wheel/2(T_fr)
  Demux/1 -> Wheel/1(T_fl)
  PAC2002/11(Mz_rl) -> Body/11(In11)
  Demux/4 -> Wheel/4(T_rr)
  PAC2002/6(Fy_fr) -> Fy_fr/1, Body/6(In6)
  Pedal/1 -> Demux/1
  [delta_fl] -> Body/13(In13)
  [delta_fr] -> Body/14(In14)
  [delta_rl] -> Body/15(In15)
  [delta_rr] -> Body/16(In16)
  Mux/1 -> Body/17(Zroad)
  Body/1(x) -> x/1
  Body/2(y) -> y/1
  Body/3(z) -> z/1
  Body/4(vx) -> vx/1, alpha_lamda/1(vx)
  Body/5(vy) -> alpha_lamda/2(vy), vy/1
  Body/6(vz) -> vz/1
  Body/7(ax) -> ax/1
  Body/8(ay) -> ay/1
  Body/9(az) -> az/1
  Body/10(roll) -> roll/1
  Body/11(phi) -> phi/1
  Body/12(yaw) -> yaw/1
  Body/13(wx) -> wx/1
  Body/16(beta_x) -> beta_x/1
  Body/14(wy) -> wy/1
  Body/15(wz) -> alpha_lamda/3(wz), wz/1
  Body/18(beta_z) -> beta_z/1
  Body/19(Fzw_fl) -> Fz_fl/1, PAC2002/9(Fz_fl), Wheel/9(Fz_fl)
  Body/20(Fzw_fr) -> Fz_fr/1, PAC2002/10(Fz_fr), Wheel/10(Fz_fr)
  Body/21(Fzw_rl) -> Fz_rl/1, Wheel/11(Fz_rl), PAC2002/11(Fz_rl)
  Body/22(Fzw_rr) -> Fz_rr/1, PAC2002/12(Fz_rr), Wheel/12(Fz_rr)
  Wheel/1(w_fl) -> w_fl/1, alpha_lamda/8(w_fl)
  Body/17(beta_y) -> beta_y/1
  Constant/1 -> Mux/1
  Constant1/1 -> Mux/2
  Constant2/1 -> Mux/3
  Constant3/1 -> Mux/4

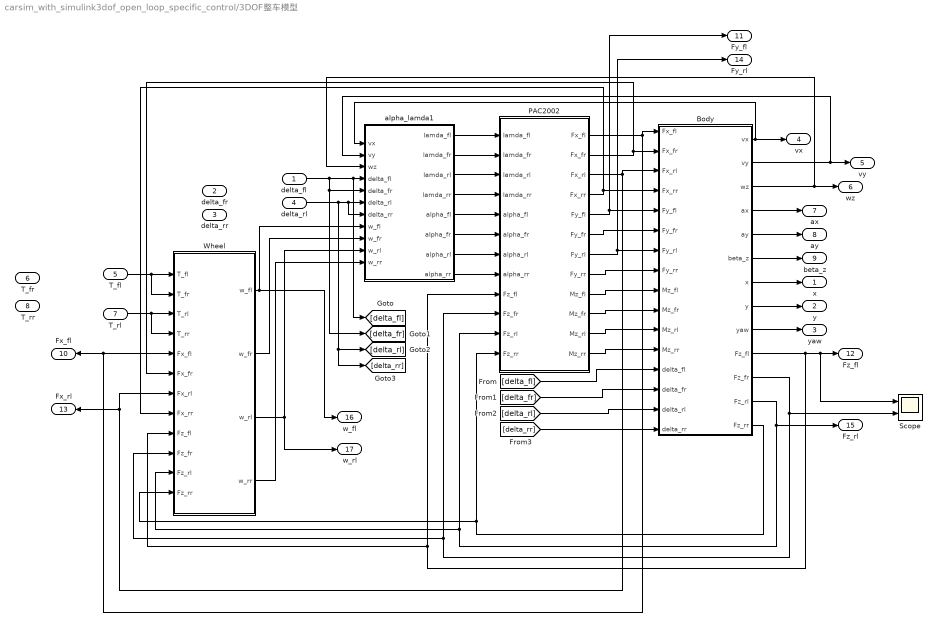
== system carsim_with_simulink3dof_open_loop_specific_control/3DOF整车模型 ==
  delta_fl : Inport
  delta_fr : Inport  Port=2
  delta_rr : Inport  Port=3
  delta_rl : Inport  Port=4
  T_fl : Inport  Port=5
  T_fr : Inport  Port=6
  T_rl : Inport  Port=7
  T_rr : Inport  Port=8
  Body : Subsystem
  PAC2002 : Subsystem
  Scope : Scope  NumInputPorts=2
  Wheel : Subsystem
  alpha_lamda1 : Subsystem
  x : Outport
  y : Outport  Port=2
  yaw : Outport  Port=3
  vx : Outport  Port=4
  vy : Outport  Port=5
  wz : Outport  Port=6
  ax : Outport  Port=7
  ay : Outport  Port=8
  beta_z : Outport  Port=9
  Fx_fl : Outport  Port=10
  Fy_fl : Outport  Port=11
  Fz_fl : Outport  Port=12
  Fx_rl : Outport  Port=13
  Fy_rl : Outport  Port=14
  Fz_rl : Outport  Port=15
  w_fl : Outport  Port=16
  w_rl : Outport  Port=17
  wires:
  PAC2002/12(Mz_rr) -> Body/12(Mz_rr)
  PAC2002/11(Mz_rl) -> Body/11(Mz_rl)
  PAC2002/10(Mz_fr) -> Body/10(Mz_fr)
  PAC2002/9(Mz_fl) -> Body/9(Mz_fl)
  T_rl/1 -> Wheel/4(T_rr), Wheel/3(T_rl)
  Body/1(vx) -> vx/1, alpha_lamda1/1(vx)
  Body/2(vy) -> vy/1, alpha_lamda1/2(vy)
  T_fl/1 -> Wheel/1(T_fl), Wheel/2(T_fr)
  Body/13(Fz_rr) -> PAC2002/12(Fz_rr), Wheel/12(Fz_rr)
  PAC2002/3(Fx_rl) -> Fx_rl/1, Wheel/7(Fx_rl), Body/3(Fx_rl)
  alpha_lamda1/6(alpha_fr) -> PAC2002/6(alpha_fr)
  Body/11(Fz_fr) -> Scope/2, PAC2002/10(Fz_fr), Wheel/10(Fz_fr)
  [delta_fr] -> Body/14(delta_fr)
  alpha_lamda1/5(alpha_fl) -> PAC2002/5(alpha_fl)
  alpha_lamda1/8(alpha_rr) -> PAC2002/8(alpha_rr)
  Wheel/3(w_rl) -> w_rl/1, alpha_lamda1/10(w_rl)
  Body/12(Fz_rl) -> Fz_rl/1, PAC2002/11(Fz_rl), Wheel/11(Fz_rl)
  alpha_lamda1/7(alpha_rl) -> PAC2002/7(alpha_rl)
  PAC2002/8(Fy_rr) -> Body/8(Fy_rr)
  alpha_lamda1/2(lamda_fr) -> PAC2002/2(lamda_fr)
  PAC2002/5(Fy_fl) -> Fy_fl/1, Body/5(Fy_fl)
  PAC2002/2(Fx_fr) -> Wheel/6(Fx_fr), Body/2(Fx_fr)
  Body/10(Fz_fl) -> Scope/1, Fz_fl/1, PAC2002/9(Fz_fl), Wheel/9(Fz_fl)
  alpha_lamda1/3(lamda_rl) -> PAC2002/3(lamda_rl)
  PAC2002/6(Fy_fr) -> Body/6(Fy_fr)
  PAC2002/7(Fy_rl) -> Fy_rl/1, Body/7(Fy_rl)
  alpha_lamda1/4(lamda_rr) -> PAC2002/4(lamda_rr)
  alpha_lamda1/1(lamda_fl) -> PAC2002/1(lamda_fl)
  PAC2002/1(Fx_fl) -> Fx_fl/1, Wheel/5(Fx_fl), Body/1(Fx_fl)
  [delta_fl] -> Body/13(delta_fl)
  Body/3(wz) -> wz/1, alpha_lamda1/3(wz)
  PAC2002/4(Fx_rr) -> Wheel/8(Fx_rr), Body/4(Fx_rr)
  Body/4(ax) -> ax/1
  Wheel/2(w_fr) -> alpha_lamda1/9(w_fr)
  Wheel/1(w_fl) -> w_fl/1, alpha_lamda1/8(w_fl)
  Wheel/4(w_rr) -> alpha_lamda1/11(w_rr)
  delta_fl/1 -> [delta_fl], alpha_lamda1/4(delta_fl), [delta_fr], alpha_lamda1/5(delta_fr)
  delta_rl/1 -> [delta_rl], [delta_rr], alpha_lamda1/7(delta_rr), alpha_lamda1/6(delta_rl)
  Body/7(x) -> x/1
  Body/8(y) -> y/1
  Body/5(ay) -> ay/1
  Body/9(yaw) -> yaw/1
  Body/6(beta_z) -> beta_z/1
  [delta_rl] -> Body/15(delta_rl)
  [delta_rr] -> Body/16(delta_rr)

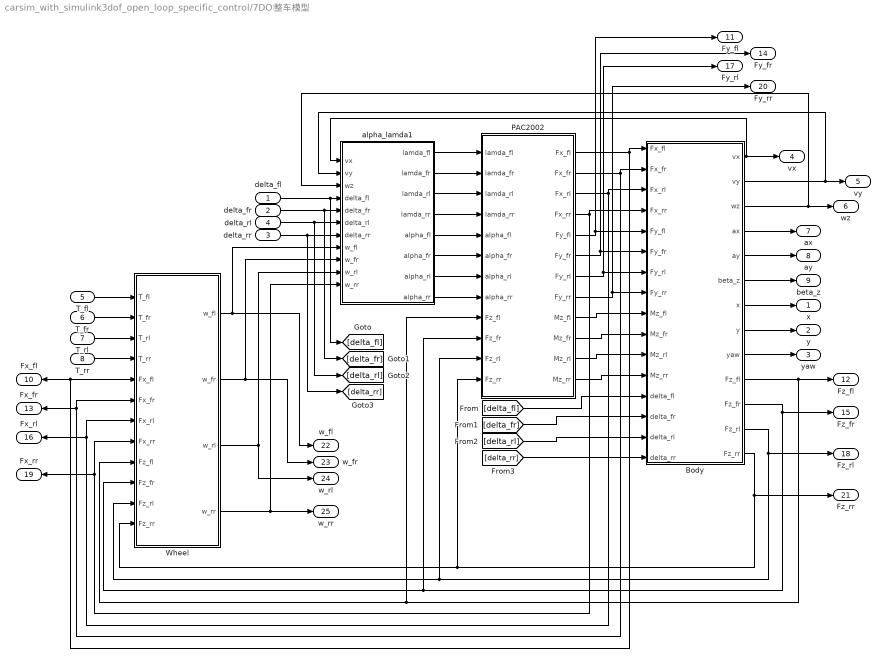
== system carsim_with_simulink3dof_open_loop_specific_control/7DOF整车模型 ==
  delta_fl : Inport
  delta_fr : Inport  Port=2
  delta_rr : Inport  Port=3
  delta_rl : Inport  Port=4
  T_fl : Inport  Port=5
  T_fr : Inport  Port=6
  T_rl : Inport  Port=7
  T_rr : Inport  Port=8
  Body : Subsystem
  PAC2002 : Subsystem
  Wheel : Subsystem
  alpha_lamda1 : Subsystem
  x : Outport
  y : Outport  Port=2
  yaw : Outport  Port=3
  vx : Outport  Port=4
  vy : Outport  Port=5
  wz : Outport  Port=6
  ax : Outport  Port=7
  ay : Outport  Port=8
  beta_z : Outport  Port=9
  Fx_fl : Outport  Port=10
  Fy_fl : Outport  Port=11
  Fz_fl : Outport  Port=12
  Fx_fr : Outport  Port=13
  Fy_fr : Outport  Port=14
  Fz_fr : Outport  Port=15
  Fx_rl : Outport  Port=16
  Fy_rl : Outport  Port=17
  Fz_rl : Outport  Port=18
  Fx_rr : Outport  Port=19
  Fy_rr : Outport  Port=20
  Fz_rr : Outport  Port=21
  w_fl : Outport  Port=22
  w_fr : Outport  Port=23
  w_rl : Outport  Port=24
  w_rr : Outport  Port=25
  wires:
  PAC2002/12(Mz_rr) -> Body/12(Mz_rr)
  PAC2002/11(Mz_rl) -> Body/11(Mz_rl)
  PAC2002/10(Mz_fr) -> Body/10(Mz_fr)
  PAC2002/9(Mz_fl) -> Body/9(Mz_fl)
  T_rr/1 -> Wheel/4(T_rr)
  T_rl/1 -> Wheel/3(T_rl)
  Body/1(vx) -> vx/1, alpha_lamda1/1(vx)
  Body/2(vy) -> vy/1, alpha_lamda1/2(vy)
  T_fl/1 -> Wheel/1(T_fl)
  Body/13(Fz_rr) -> PAC2002/12(Fz_rr), Wheel/12(Fz_rr), Fz_rr/1
  T_fr/1 -> Wheel/2(T_fr)
  PAC2002/3(Fx_rl) -> Fx_rl/1, Wheel/7(Fx_rl), Body/3(Fx_rl)
  alpha_lamda1/6(alpha_fr) -> PAC2002/6(alpha_fr)
  Body/11(Fz_fr) -> Fz_fr/1, PAC2002/10(Fz_fr), Wheel/10(Fz_fr)
  [delta_fr] -> Body/14(delta_fr)
  alpha_lamda1/5(alpha_fl) -> PAC2002/5(alpha_fl)
  alpha_lamda1/8(alpha_rr) -> PAC2002/8(alpha_rr)
  Wheel/3(w_rl) -> w_rl/1, alpha_lamda1/10(w_rl)
  Body/12(Fz_rl) -> Fz_rl/1, PAC2002/11(Fz_rl), Wheel/11(Fz_rl)
  alpha_lamda1/7(alpha_rl) -> PAC2002/7(alpha_rl)
  PAC2002/8(Fy_rr) -> Fy_rr/1, Body/8(Fy_rr)
  alpha_lamda1/2(lamda_fr) -> PAC2002/2(lamda_fr)
  PAC2002/5(Fy_fl) -> Fy_fl/1, Body/5(Fy_fl)
  PAC2002/2(Fx_fr) -> Fx_fr/1, Wheel/6(Fx_fr), Body/2(Fx_fr)
  Body/10(Fz_fl) -> Fz_fl/1, PAC2002/9(Fz_fl), Wheel/9(Fz_fl)
  alpha_lamda1/3(lamda_rl) -> PAC2002/3(lamda_rl)
  PAC2002/6(Fy_fr) -> Fy_fr/1, Body/6(Fy_fr)
  PAC2002/7(Fy_rl) -> Fy_rl/1, Body/7(Fy_rl)
  alpha_lamda1/4(lamda_rr) -> PAC2002/4(lamda_rr)
  alpha_lamda1/1(lamda_fl) -> PAC2002/1(lamda_fl)
  PAC2002/1(Fx_fl) -> Fx_fl/1, Wheel/5(Fx_fl), Body/1(Fx_fl)
  [delta_fl] -> Body/13(delta_fl)
  Body/3(wz) -> wz/1, alpha_lamda1/3(wz)
  PAC2002/4(Fx_rr) -> Fx_rr/1, Wheel/8(Fx_rr), Body/4(Fx_rr)
  Body/4(ax) -> ax/1
  Wheel/2(w_fr) -> w_fr/1, alpha_lamda1/9(w_fr)
  Wheel/1(w_fl) -> w_fl/1, alpha_lamda1/8(w_fl)
  Wheel/4(w_rr) -> w_rr/1, alpha_lamda1/11(w_rr)
  delta_fl/1 -> [delta_fl], alpha_lamda1/4(delta_fl)
  delta_fr/1 -> alpha_lamda1/5(delta_fr), [delta_fr]
  delta_rl/1 -> [delta_rl], alpha_lamda1/6(delta_rl)
  delta_rr/1 -> alpha_lamda1/7(delta_rr), [delta_rr]
  Body/7(x) -> x/1
  Body/8(y) -> y/1
  Body/5(ay) -> ay/1
  Body/9(yaw) -> yaw/1
  Body/6(beta_z) -> beta_z/1
  [delta_rl] -> Body/15(delta_rl)
  [delta_rr] -> Body/16(delta_rr)

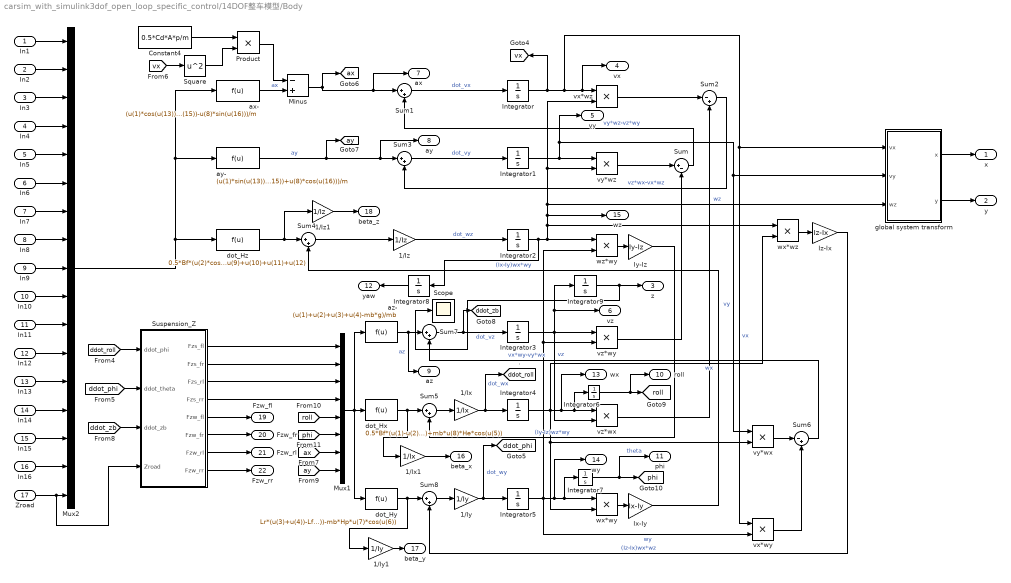
== system carsim_with_simulink3dof_open_loop_specific_control/14DOF整车模型/Body ==
  In1 : Inport
  In2 : Inport  Port=2
  In3 : Inport  Port=3
  In4 : Inport  Port=4
  In5 : Inport  Port=5
  In6 : Inport  Port=6
  In7 : Inport  Port=7
  In8 : Inport  Port=8
  In9 : Inport  Port=9
  In10 : Inport  Port=10
  In11 : Inport  Port=11
  In12 : Inport  Port=12
  In13 : Inport  Port=13
  In14 : Inport  Port=14
  In15 : Inport  Port=15
  In16 : Inport  Port=16
  Zroad : Inport  Port=17
  1/Ix : Gain  Gain=1/Ix
  1/Ix1 : Gain  Gain=1/Ix
  1/Iy : Gain  Gain=1/Iy
  1/Iy1 : Gain  Gain=1/Iy
  1/Iz : Gain  Gain=1/Iz
  1/Iz1 : Gain  Gain=1/Iz
  Constant4 : Constant  Value=0.5*Cd*A*p/m
  Integrator : Integrator  InitialCondition=vx0  LimitOutput=on  LowerSaturationLimit=0
  Integrator1 : Integrator  InitialCondition=vy0
  Integrator2 : Integrator  InitialCondition=wz0
  Integrator{3..6,8} (5 alike) : Integrator
  Integrator7 : Integrator  InitialCondition=1.2245e-3
  Integrator9 : Integrator  InitialCondition=-0.131
  Ix-Iy : Gain  Gain=Ix-Iy
  Iy-Iz : Gain  Gain=Iy-Iz
  Iz-Ix : Gain  Gain=Iz-Ix
  Minus : Sum  Inputs=-+
  Mux1 : Mux  Inputs=8
  Mux2 : Mux  Inputs=17
  Product : Product
  Scope : Scope
  Square : Math  Operator=square
  Sum : Sum  Inputs=|+-
  Sum{1,3..5,7..8} (6 alike) : Sum  Inputs=|++
  Sum2 : Sum  Inputs=|-+
  Sum6 : Sum  Inputs=|-+
  Suspension_Z : Subsystem
  ax- : Fcn  Expr="(u(1)*cos(u(13))+u(2)*cos(u(14))-u(5)*sin(u(13))-u(6)*sin(u(14))+   u(3)*cos(u(15))+u(4)*cos(u(16))-u(7)*sin(u(15))-u(8)*sin(u(16)))/m"
  ay- : Fcn  Expr=(u(1)*sin(u(13))+u(2)*sin(u(14))+u(5)*cos(u(13))+u(6)*cos(u(14))+u(3)*sin(u(15))+u(4)*sin(u(16))+u(7)*cos(u(15))+u(8)*cos(u(16)))/m
  az- : Fcn  Expr=(u(1)+u(2)+u(3)+u(4)-mb*g)/mb
  dot_Hx : Fcn  Expr=0.5*Bf*(u(1)-u(2))+0.5*Br*(u(3)-u(4))+mb*g*He*sin(u(5))+mb*u(8)*He*cos(u(5))
  dot_Hy : Fcn  Expr=Lr*(u(3)+u(4))-Lf*(u(1)+u(2))+mb*g*Hp*sin(u(6))-mb*Hp*u(7)*cos(u(6))
  dot_Hz : Fcn  Expr=0.5*Bf*(u(2)*cos(u(14))-u(1)*cos(u(13))-u(6)*sin(u(14))+u(5)*sin(u(13)))+0.5*Br*(u(4)*cos(u(16))-u(3)*cos(u(15))-u(8)*sin(u(16))+u(7)*sin(u(15)))+Lf*(u(1)*sin(u(13))+u(5)*cos(u(13))+u(2)*sin(u(14))+u(6)*cos(u(14)))-Lr*(u(3)*sin(u(15))+u(7)*cos(u(15))+u(4)*sin(u(16))+u(8)*cos(u(16)))+u(9)+u(10)+u(11)+u(12)
  global system transform : Subsystem
  vx*wy : Product
  vx*wz : Product
  vy*wx : Product
  vy*wz : Product
  vz*wx : Product
  vz*wy : Product
  wx*wy : Product
  wx*wz : Product
  wz*wy : Product
  x : Outport
  y : Outport  Port=2
  z : Outport  Port=3
  vx : Outport  Port=4
  vy : Outport  Port=5
  vz : Outport  Port=6
  ax : Outport  Port=7
  ay : Outport  Port=8
  az : Outport  Port=9
  roll : Outport  Port=10
  phi : Outport  Port=11
  yaw : Outport  Port=12
  wx : Outport  Port=13
  wy : Outport  Port=14
  wz : Outport  Port=15
  beta_x : Outport  Port=16
  beta_y : Outport  Port=17
  beta_z : Outport  Port=18
  Fzw_fl : Outport  Port=19
  Fzw_fr : Outport  Port=20
  Fzw_rl : Outport  Port=21
  Fzw_rr : Outport  Port=22
  tag scope: ax=global, ay=global, ddot_phi=global, ddot_roll=global, ddot_zb=global, phi=global, roll=global, vx=global
  wires:
  ay-/1 -> [ay], ay/1, Sum3/1  "ay"
  vx*wz/1 -> Sum2/1
  Integrator/1 -> vx*wy/1, global system transform/1(vx), vx/1, vx*wz/1, [vx]  "vx"
  Suspension_Z/3(Fzs_rl) -> Mux1/3
  [phi] -> Mux1/6
  vy*wx/1 -> Sum6/1
  wz*wy/1 -> Iy-Iz/1
  vy*wz/1 -> Sum/1
  Integrator5/1 -> wy/1, wx*wy/1, Integrator7/1, wz*wy/2, vz*wy/2, vx*wy/2  "wy"
  Sum7/1 -> Integrator3/1, [ddot_zb]  "dot_vz"
  Integrator2/1 -> Integrator8/1, wz*wy/1, wz/1, vx*wz/2, vy*wz/2, global system transform/3(wz), wx*wz/1  "wz"
  az-/1 -> Sum7/1, az/1  "az"
  dot_Hz/1 -> 1/Iz1/1, Sum4/1
  vx*wy/1 -> Sum6/2
  vz*wx/1 -> Sum2/2
  Integrator3/1 -> vz*wy/1, vz*wx/2, vz/1, Integrator9/1  "vz"
  Mux1/1 -> az-/1, dot_Hx/1, dot_Hy/1
  Minus/1 -> ax/1, Sum1/1, [ax]
  dot_Hy/1 -> 1/Iy1/1, Sum8/1
  Mux2/1 -> ax-/1, ay-/1, dot_Hz/1
  In5/1 -> Mux2/5
  global system transform/1(x) -> x/1
  [ddot_roll] -> Suspension_Z/1(ddot_phi)
  Integrator1/1 -> vy*wz/1, vy/1, vy*wx/1, global system transform/2(vy)  "vy"
  Suspension_Z/7(Fzw_rl) -> Fzw_rl/1
  1/Ix/1 -> Integrator4/1, [ddot_roll]  "dot_wx"
  1/Iy/1 -> Integrator5/1, [ddot_phi]  "dot_wy"
  wx*wy/1 -> Ix-Iy/1
  Integrator7/1 -> phi/1, [phi]  "theta"
  Square/1 -> Product/2
  1/Iz/1 -> Integrator2/1  "dot_wz"
  Sum/1 -> Sum1/2  "vy*wz-vz*wy"
  Zroad/1 -> Suspension_Z/4(Zroad), Mux2/17
  Integrator4/1 -> wx/1, vz*wx/1, Integrator6/1, wx*wy/2, vy*wx/2, wx*wz/2  "wx"
  Sum2/1 -> Sum3/2  "vz*wx-vx*wz"
  Suspension_Z/6(Fzw_fr) -> Fzw_fr/1
  In12/1 -> Mux2/12
  Sum3/1 -> Integrator1/1  "dot_vy"
  wx*wz/1 -> Iz-Ix/1
  Sum6/1 -> Sum7/2  "vx*wy-vy*wx"
  In16/1 -> Mux2/16
  [ay] -> Mux1/8
  [vx] -> Square/1
  [ddot_zb] -> Suspension_Z/3(ddot_zb)
  Product/1 -> Minus/1
  Ix-Iy/1 -> Sum4/2  "(Ix-Iy)wx*wy"
  In2/1 -> Mux2/2
  Iz-Ix/1 -> Sum8/2  "(Iz-Ix)wx*wz"
  Sum4/1 -> 1/Iz/1
  Suspension_Z/2(Fzs_fr) -> Mux1/2
  Integrator6/1 -> roll/1, [roll]
  Sum5/1 -> 1/Ix/1
  dot_Hx/1 -> 1/Ix1/1, Sum5/1
  Sum8/1 -> 1/Iy/1
  ax-/1 -> Minus/2  "ax"
  Iy-Iz/1 -> Sum5/2  "(Iy-Iz)wz*wy"
  [ddot_phi] -> Suspension_Z/2(ddot_theta)
  Constant4/1 -> Product/1
  vz*wy/1 -> Sum/2
  Suspension_Z/4(Fzs_rr) -> Mux1/4
  In6/1 -> Mux2/6
  [roll] -> Mux1/5
  Suspension_Z/1(Fzs_fl) -> Mux1/1
  Sum1/1 -> Integrator/1  "dot_vx"
  Suspension_Z/8(Fzw_rr) -> Fzw_rr/1
  [ax] -> Mux1/7
  In14/1 -> Mux2/14
  In11/1 -> Mux2/11
  In3/1 -> Mux2/3
  Suspension_Z/5(Fzw_fl) -> Fzw_fl/1
  Integrator8/1 -> yaw/1
  In1/1 -> Mux2/1
  In10/1 -> Mux2/10
  In4/1 -> Mux2/4
  In15/1 -> Mux2/15
  global system transform/2(y) -> y/1
  Integrator9/1 -> Scope/1, z/1
  In8/1 -> Mux2/8
  In13/1 -> Mux2/13
  In9/1 -> Mux2/9
  In7/1 -> Mux2/7
  1/Iz1/1 -> beta_z/1
  1/Ix1/1 -> beta_x/1
  1/Iy1/1 -> beta_y/1

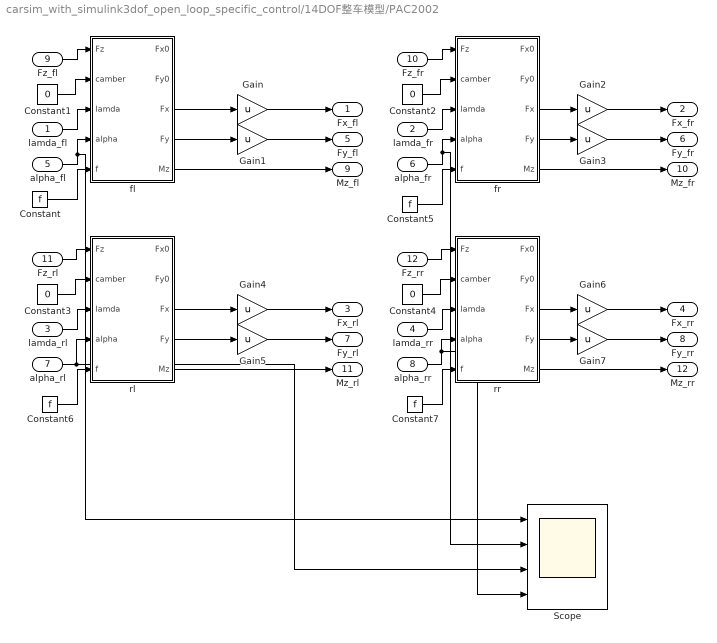
== system carsim_with_simulink3dof_open_loop_specific_control/14DOF整车模型/PAC2002 ==
  lamda_fl : Inport
  lamda_fr : Inport  Port=2
  lamda_rl : Inport  Port=3
  lamda_rr : Inport  Port=4
  alpha_fl : Inport  Port=5
  alpha_fr : Inport  Port=6
  alpha_rl : Inport  Port=7
  alpha_rr : Inport  Port=8
  Fz_fl : Inport  Port=9
  Fz_fr : Inport  Port=10
  Fz_rl : Inport  Port=11
  Fz_rr : Inport  Port=12
  Constant{,5..7} (4 alike) : Constant  Value=f
  Constant{1..4} (4 alike) : Constant  Value=0
  Gain{,1..7} (8 alike) : Gain  Gain=u
  Scope : Scope  NumInputPorts=4
  fl : MATLAB Function  TreatAsAtomicUnit=on
  fr : MATLAB Function  TreatAsAtomicUnit=on
  rl : MATLAB Function  TreatAsAtomicUnit=on
  rr : MATLAB Function  TreatAsAtomicUnit=on
  Fx_fl : Outport
  Fx_fr : Outport  Port=2
  Fx_rl : Outport  Port=3
  Fx_rr : Outport  Port=4
  Fy_fl : Outport  Port=5
  Fy_fr : Outport  Port=6
  Fy_rl : Outport  Port=7
  Fy_rr : Outport  Port=8
  Mz_fl : Outport  Port=9
  Mz_fr : Outport  Port=10
  Mz_rl : Outport  Port=11
  Mz_rr : Outport  Port=12
  wires:
  Constant4/1 -> rr/2(camber)
  Constant3/1 -> rl/2(camber)
  Constant2/1 -> fr/2(camber)
  rr/5(Mz) -> Mz_rr/1
  rl/5(Mz) -> Mz_rl/1
  Fz_rr/1 -> rr/1(Fz)
  alpha_rr/1 -> Scope/4, rr/4(alpha)
  lamda_rr/1 -> rr/3(lamda)
  Fz_rl/1 -> rl/1(Fz)
  alpha_rl/1 -> Scope/3, rl/4(alpha)
  lamda_rl/1 -> rl/3(lamda)
  fr/5(Mz) -> Mz_fr/1
  Fz_fr/1 -> fr/1(Fz)
  alpha_fr/1 -> Scope/2, fr/4(alpha)
  lamda_fr/1 -> fr/3(lamda)
  fl/5(Mz) -> Mz_fl/1
  Constant1/1 -> fl/2(camber)
  Fz_fl/1 -> fl/1(Fz)
  alpha_fl/1 -> Scope/1, fl/4(alpha)
  lamda_fl/1 -> fl/3(lamda)
  fl/3(Fx) -> Gain/1
  fl/4(Fy) -> Gain1/1
  fr/4(Fy) -> Gain3/1
  rr/3(Fx) -> Gain6/1
  rr/4(Fy) -> Gain7/1
  rl/3(Fx) -> Gain4/1
  rl/4(Fy) -> Gain5/1
  fr/3(Fx) -> Gain2/1
  Gain/1 -> Fx_fl/1
  Gain1/1 -> Fy_fl/1
  Gain2/1 -> Fx_fr/1
  Gain3/1 -> Fy_fr/1
  Gain4/1 -> Fx_rl/1
  Gain5/1 -> Fy_rl/1
  Gain6/1 -> Fx_rr/1
  Gain7/1 -> Fy_rr/1
  Constant/1 -> fl/5(f)
  Constant5/1 -> fr/5(f)
  Constant6/1 -> rl/5(f)
  Constant7/1 -> rr/5(f)

== system carsim_with_simulink3dof_open_loop_specific_control/14DOF整车模型/Wheel ==
  T_fl : Inport
  T_fr : Inport  Port=2
  T_rl : Inport  Port=3
  T_rr : Inport  Port=4
  Fx_fl : Inport  Port=5
  Fx_fr : Inport  Port=6
  Fx_rl : Inport  Port=7
  Fx_rr : Inport  Port=8
  Fz_fl : Inport  Port=9
  Fz_fr : Inport  Port=10
  Fz_rl : Inport  Port=11
  Fz_rr : Inport  Port=12
  fl : Subsystem
  fr : Subsystem
  rl : Subsystem
  rr : Subsystem
  w_fl : Outport
  w_fr : Outport  Port=2
  w_rl : Outport  Port=3
  w_rr : Outport  Port=4
  wires:
  rr/1(w_rr) -> w_rr/1
  Fz_rr/1 -> rr/3(Fz_rr)
  Fx_rr/1 -> rr/2(Fx_rr)
  T_rr/1 -> rr/1(T_rr)
  rl/1(w_rl) -> w_rl/1
  Fz_rl/1 -> rl/3(Fz_rl)
  Fx_rl/1 -> rl/2(Fx_rl)
  T_rl/1 -> rl/1(T_rl)
  Fz_fr/1 -> fr/3(Fz_fr)
  Fx_fr/1 -> fr/2(Fx_fr)
  T_fr/1 -> fr/1(T_fr)
  fr/1(w_fr) -> w_fr/1
  fl/1(w_fl) -> w_fl/1
  Fz_fl/1 -> fl/3(Fz_fl)
  Fx_fl/1 -> fl/2(Fx_fl)
  T_fl/1 -> fl/1(T_fl)

== system carsim_with_simulink3dof_open_loop_specific_control/14DOF整车模型/alpha_lamda ==
  vx : Inport
  vy : Inport  Port=2
  wz : Inport  Port=3
  delta_fl : Inport  Port=4
  delta_fr : Inport  Port=5
  delta_rl : Inport  Port=6
  delta_rr : Inport  Port=7
  w_fl : Inport  Port=8
  w_fr : Inport  Port=9
  w_rl : Inport  Port=10
  w_rr : Inport  Port=11
  alpha : Subsystem
  lamda : Subsystem
  lamda_fl : Outport
  lamda_fr : Outport  Port=2
  lamda_rl : Outport  Port=3
  lamda_rr : Outport  Port=4
  alpha_fl : Outport  Port=5
  alpha_fr : Outport  Port=6
  alpha_rl : Outport  Port=7
  alpha_rr : Outport  Port=8
  wires:
  alpha/1(alpha_fl) -> alpha_fl/1
  alpha/2(alpha_fr) -> alpha_fr/1
  alpha/3(alpha_rl) -> alpha_rl/1
  alpha/4(alpha_rr) -> alpha_rr/1
  vx/1 -> lamda/1(vx), alpha/1(vx)
  vy/1 -> lamda/2(vy), alpha/2(vy)
  wz/1 -> lamda/3(wz), alpha/3(wz)
  delta_fl/1 -> lamda/4(delta_fl), alpha/4(delta_fl)
  delta_fr/1 -> lamda/5(delta_fr), alpha/5(delta_fr)
  w_fl/1 -> lamda/6(w_fl)
  w_fr/1 -> lamda/7(w_fr)
  w_rl/1 -> lamda/8(w_rl)
  w_rr/1 -> lamda/9(w_rr)
  lamda/1(lamda_fl) -> lamda_fl/1
  lamda/2(lamda_fr) -> lamda_fr/1
  lamda/4(lamda_rr) -> lamda_rr/1
  lamda/3(lamda_rl) -> lamda_rl/1
  delta_rl/1 -> lamda/10(delta_rl), alpha/6(delta_rl)
  delta_rr/1 -> lamda/11(delta_rr), alpha/7(delta_rr)

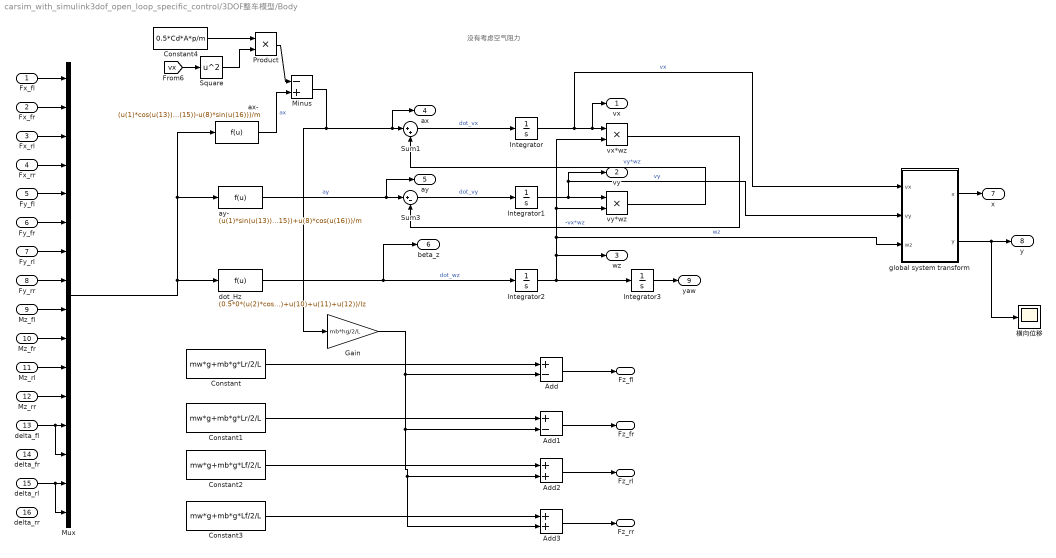
== system carsim_with_simulink3dof_open_loop_specific_control/3DOF整车模型/Body ==
  note: 没有考虑空气阻力
  Fx_fl : Inport
  Fx_fr : Inport  Port=2
  Fx_rl : Inport  Port=3
  Fx_rr : Inport  Port=4
  Fy_fl : Inport  Port=5
  Fy_fr : Inport  Port=6
  Fy_rl : Inport  Port=7
  Fy_rr : Inport  Port=8
  Mz_fl : Inport  Port=9
  Mz_fr : Inport  Port=10
  Mz_rl : Inport  Port=11
  Mz_rr : Inport  Port=12
  delta_fl : Inport  Port=13
  delta_fr : Inport  Port=14
  delta_rl : Inport  Port=15
  delta_rr : Inport  Port=16
  Add : Sum  Inputs=+-
  Add1 : Sum  Inputs=+-
  Add2 : Sum
  Add3 : Sum
  Constant : Constant  Value=mw*g+mb*g*Lr/2/L
  Constant1 : Constant  Value=mw*g+mb*g*Lr/2/L
  Constant2 : Constant  Value=mw*g+mb*g*Lf/2/L
  Constant3 : Constant  Value=mw*g+mb*g*Lf/2/L
  Constant4 : Constant  Value=0.5*Cd*A*p/m
  Gain : Gain  Gain=mb*hg/2/L
  Integrator : Integrator  InitialCondition=vx0  LimitOutput=on  LowerSaturationLimit=0
  Integrator1 : Integrator  InitialCondition=vy0
  Integrator2 : Integrator  InitialCondition=wz0
  Integrator3 : Integrator
  Minus : Sum  Inputs=-+
  Mux : Mux  Inputs=16
  Product : Product
  Square : Math  Operator=square
  Sum1 : Sum  Inputs=|++
  Sum3 : Sum  Inputs=|+-
  ax- : Fcn  Expr=(u(1)*cos(u(13))+u(2)*cos(u(14))-u(5)*sin(u(13))-u(6)*sin(u(14))+u(3)*cos(u(15))+u(4)*cos(u(16))-u(7)*sin(u(15))-u(8)*sin(u(16)))/m
  ay- : Fcn  Expr=(u(1)*sin(u(13))+u(2)*sin(u(14))+u(5)*cos(u(13))+u(6)*cos(u(14))+u(3)*sin(u(15))+u(4)*sin(u(16))+u(7)*cos(u(15))+u(8)*cos(u(16)))/m
  dot_Hz : Fcn  Expr=(0.5*0*(u(2)*cos(u(14))-u(1)*cos(u(13))-u(6)*sin(u(14))+u(5)*sin(u(13)))+0.5*0*(u(4)*cos(u(16))-u(3)*cos(u(15))-u(8)*sin(u(16))+u(7)*sin(u(15)))+Lf*(u(1)*sin(u(13))+u(5)*cos(u(13))+u(2)*sin(u(14))+u(6)*cos(u(14)))-Lr*(u(3)*sin(u(15))+u(7)*cos(u(15))+u(4)*sin(u(16))+u(8)*cos(u(16)))+u(9)+u(10)+u(11)+u(12))/Iz
  global system transform : Subsystem
  vx*wz : Product
  vy*wz : Product
  横向位移 : Scope
  vx : Outport
  vy : Outport  Port=2
  wz : Outport  Port=3
  ax : Outport  Port=4
  ay : Outport  Port=5
  beta_z : Outport  Port=6
  x : Outport  Port=7
  y : Outport  Port=8
  yaw : Outport  Port=9
  Fz_fl : Outport  Port=10
  Fz_fr : Outport  Port=11
  Fz_rl : Outport  Port=12
  Fz_rr : Outport  Port=13
  wires:
  global system transform/2(y) -> y/1, 横向位移/1
  global system transform/1(x) -> x/1
  Mux/1 -> dot_Hz/1, ay-/1, ax-/1
  delta_fl/1 -> Mux/14, Mux/13
  Mz_rr/1 -> Mux/12
  Mz_rl/1 -> Mux/11
  Mz_fr/1 -> Mux/10
  Mz_fl/1 -> Mux/9
  Fy_rr/1 -> Mux/8
  Fy_rl/1 -> Mux/7
  Fy_fr/1 -> Mux/6
  Fy_fl/1 -> Mux/5
  Fx_rr/1 -> Mux/4
  Fx_rl/1 -> Mux/3
  Fx_fr/1 -> Mux/2
  Fx_fl/1 -> Mux/1
  Sum1/1 -> Integrator/1  "dot_vx"
  Integrator/1 -> vx/1, vx*wz/1, global system transform/1(vx)  "vx"
  Integrator1/1 -> global system transform/2(vy), vy/1, vy*wz/1  "vy"
  Sum3/1 -> Integrator1/1  "dot_vy"
  dot_Hz/1 -> beta_z/1, Integrator2/1  "dot_wz"
  Integrator2/1 -> Integrator3/1, global system transform/3(wz), vy*wz/2, vx*wz/2, wz/1  "wz"
  ay-/1 -> ay/1, Sum3/1  "ay"
  vy*wz/1 -> Sum1/2  "vy*wz"
  vx*wz/1 -> Sum3/2  "-vx*wz"
  Constant/1 -> Add/1
  Gain/1 -> Add3/2, Add2/2, Add1/2, Add/2
  Add/1 -> Fz_fl/1
  Constant1/1 -> Add1/1
  Add1/1 -> Fz_fr/1
  Constant2/1 -> Add2/1
  Add2/1 -> Fz_rl/1
  Constant3/1 -> Add3/1
  Add3/1 -> Fz_rr/1
  Constant4/1 -> Product/1
  Square/1 -> Product/2
  [vx] -> Square/1
  Product/1 -> Minus/1
  ax-/1 -> Minus/2  "ax"
  Minus/1 -> Gain/1, ax/1, Sum1/1
  delta_rl/1 -> Mux/16, Mux/15
  Integrator3/1 -> yaw/1

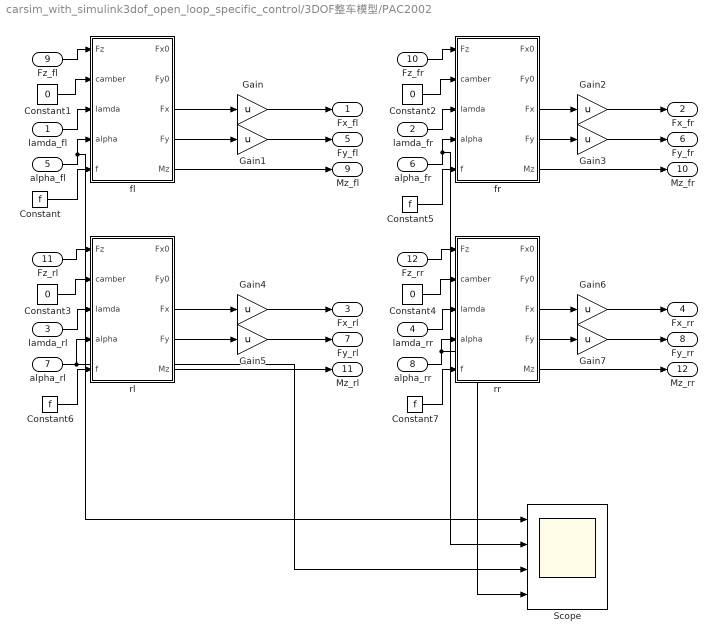
== system carsim_with_simulink3dof_open_loop_specific_control/3DOF整车模型/PAC2002 ==
  lamda_fl : Inport
  lamda_fr : Inport  Port=2
  lamda_rl : Inport  Port=3
  lamda_rr : Inport  Port=4
  alpha_fl : Inport  Port=5
  alpha_fr : Inport  Port=6
  alpha_rl : Inport  Port=7
  alpha_rr : Inport  Port=8
  Fz_fl : Inport  Port=9
  Fz_fr : Inport  Port=10
  Fz_rl : Inport  Port=11
  Fz_rr : Inport  Port=12
  Constant{,5..7} (4 alike) : Constant  Value=f
  Constant{1..4} (4 alike) : Constant  Value=0
  Gain{,1..7} (8 alike) : Gain  Gain=u
  Scope : Scope  NumInputPorts=4
  fl : MATLAB Function  TreatAsAtomicUnit=on
  fr : MATLAB Function  TreatAsAtomicUnit=on
  rl : MATLAB Function  TreatAsAtomicUnit=on
  rr : MATLAB Function  TreatAsAtomicUnit=on
  Fx_fl : Outport
  Fx_fr : Outport  Port=2
  Fx_rl : Outport  Port=3
  Fx_rr : Outport  Port=4
  Fy_fl : Outport  Port=5
  Fy_fr : Outport  Port=6
  Fy_rl : Outport  Port=7
  Fy_rr : Outport  Port=8
  Mz_fl : Outport  Port=9
  Mz_fr : Outport  Port=10
  Mz_rl : Outport  Port=11
  Mz_rr : Outport  Port=12
  wires:
  Constant4/1 -> rr/2(camber)
  Constant3/1 -> rl/2(camber)
  Constant2/1 -> fr/2(camber)
  rr/5(Mz) -> Mz_rr/1
  rl/5(Mz) -> Mz_rl/1
  Fz_rr/1 -> rr/1(Fz)
  alpha_rr/1 -> Scope/4, rr/4(alpha)
  lamda_rr/1 -> rr/3(lamda)
  Fz_rl/1 -> rl/1(Fz)
  alpha_rl/1 -> Scope/3, rl/4(alpha)
  lamda_rl/1 -> rl/3(lamda)
  fr/5(Mz) -> Mz_fr/1
  Fz_fr/1 -> fr/1(Fz)
  alpha_fr/1 -> Scope/2, fr/4(alpha)
  lamda_fr/1 -> fr/3(lamda)
  fl/5(Mz) -> Mz_fl/1
  Constant1/1 -> fl/2(camber)
  Fz_fl/1 -> fl/1(Fz)
  alpha_fl/1 -> Scope/1, fl/4(alpha)
  lamda_fl/1 -> fl/3(lamda)
  fl/3(Fx) -> Gain/1
  fl/4(Fy) -> Gain1/1
  fr/4(Fy) -> Gain3/1
  rr/3(Fx) -> Gain6/1
  rr/4(Fy) -> Gain7/1
  rl/3(Fx) -> Gain4/1
  rl/4(Fy) -> Gain5/1
  fr/3(Fx) -> Gain2/1
  Gain/1 -> Fx_fl/1
  Gain1/1 -> Fy_fl/1
  Gain2/1 -> Fx_fr/1
  Gain3/1 -> Fy_fr/1
  Gain4/1 -> Fx_rl/1
  Gain5/1 -> Fy_rl/1
  Gain6/1 -> Fx_rr/1
  Gain7/1 -> Fy_rr/1
  Constant/1 -> fl/5(f)
  Constant5/1 -> fr/5(f)
  Constant6/1 -> rl/5(f)
  Constant7/1 -> rr/5(f)

== system carsim_with_simulink3dof_open_loop_specific_control/3DOF整车模型/Wheel ==
  T_fl : Inport
  T_fr : Inport  Port=2
  T_rl : Inport  Port=3
  T_rr : Inport  Port=4
  Fx_fl : Inport  Port=5
  Fx_fr : Inport  Port=6
  Fx_rl : Inport  Port=7
  Fx_rr : Inport  Port=8
  Fz_fl : Inport  Port=9
  Fz_fr : Inport  Port=10
  Fz_rl : Inport  Port=11
  Fz_rr : Inport  Port=12
  fl : Subsystem
  fr : Subsystem
  rl : Subsystem
  rr : Subsystem
  w_fl : Outport
  w_fr : Outport  Port=2
  w_rl : Outport  Port=3
  w_rr : Outport  Port=4
  wires:
  T_fl/1 -> fl/1(T_fl)
  Fx_fl/1 -> fl/2(Fx_fl)
  Fz_fl/1 -> fl/3(Fz_fl)
  fl/1(w_fl) -> w_fl/1
  fr/1(w_fr) -> w_fr/1
  T_fr/1 -> fr/1(T_fr)
  Fx_fr/1 -> fr/2(Fx_fr)
  Fz_fr/1 -> fr/3(Fz_fr)
  T_rl/1 -> rl/1(T_rl)
  Fx_rl/1 -> rl/2(Fx_rl)
  Fz_rl/1 -> rl/3(Fz_rl)
  rl/1(w_rl) -> w_rl/1
  T_rr/1 -> rr/1(T_rr)
  Fx_rr/1 -> rr/2(Fx_rr)
  Fz_rr/1 -> rr/3(Fz_rr)
  rr/1(w_rr) -> w_rr/1
